simulink model "asbCubeSatVehicleOperator"  (R2025b)
settings: Solver=VariableStepAuto  StartTime=0.0  StopTime=10.0  RelTol=1e-3
undefined symbols (not defined in the file): CubeSatTimeStep
libraries: simulink x1
settings Model: DataDictionary=asbCubeSatArchInterfaceData.sldd  Creator=The MathWorks, Inc.  LastModifiedBy=The MathWorks, Inc.
settings SolverCC: AlgebraicLoopSolver=TrustRegion  MaxZcPerStep=1.0
settings DebuggingCC: UnconnectedInputMsg=warning  UnconnectedOutputMsg=warning  UnconnectedLineMsg=warning
settings ModelReferenceCC: EnableRefExpFcnMdlSchedulingChecks=on
settings RTWCC: GPUComputeCapability=3.5  DLArmComputeVersion=19.05

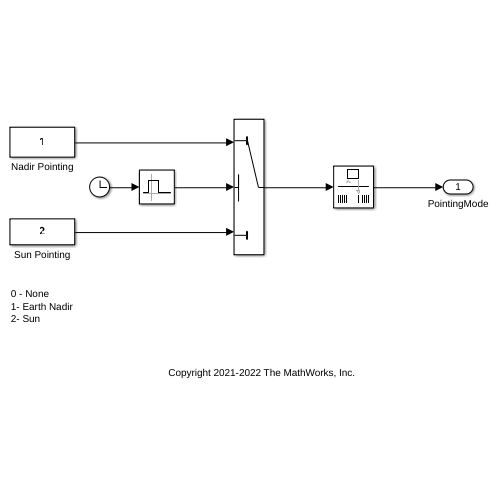
[thumbnail: Simulink's stored preview of the top-level diagram]
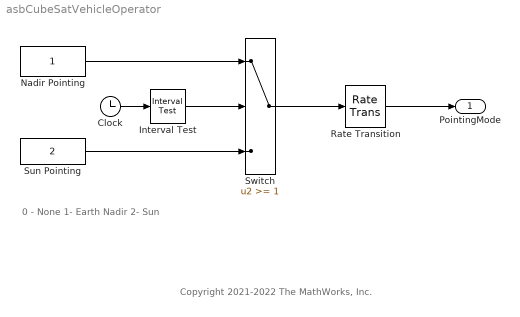
== system asbCubeSatVehicleOperator ==
  note: Copyright 2021-2022 The MathWorks, Inc.
  note: 0 - None
      | 1- Earth Nadir
      | 2- Sun
  Clock : Clock
  Interval Test : simulink/Logic and Bit Operations/Interval Test  IntervalClosedRight=on  uplimit=8200  IntervalClosedLeft=on  lowlimit=7500  OutDataTypeStr=boolean
  Nadir Pointing : Constant  SampleTime=CubeSatTimeStep
  Rate Transition : RateTransition  OutPortSampleTime=CubeSatTimeStep
  Sun Pointing : Constant  Value=2  SampleTime=CubeSatTimeStep
  Switch : Switch  Threshold=1  SaturateOnIntegerOverflow=off  InputSameDT=off
  PointingMode : Outport
  wires:
  Clock/1 -> Interval Test/1
  Interval Test/1 -> Switch/2
  Nadir Pointing/1 -> Switch/1
  Sun Pointing/1 -> Switch/3
  Switch/1 -> Rate Transition/1
  Rate Transition/1 -> PointingMode/1
